simulink model "rocket_multiphase"  (R2024b)
settings: Solver=VariableStepAuto  StartTime=0.0  StopTime=40  RelTol=1e-3
undefined symbols (not defined in the file): K, Kd, Ki, Kp, Tf
libraries: simulink x1, slpidlib x1
settings Model: Creator=fpigh  LastModifiedBy=fpigh

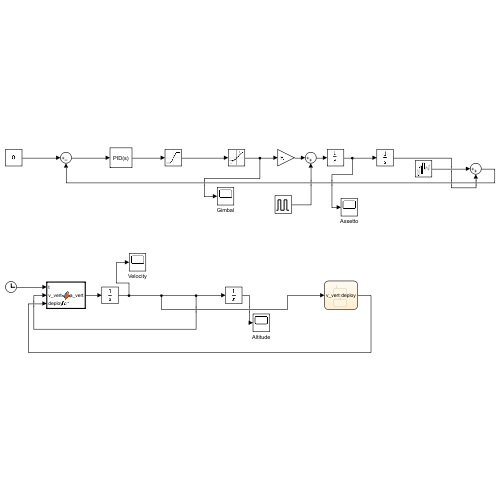
[thumbnail: Simulink's stored preview of the top-level diagram]
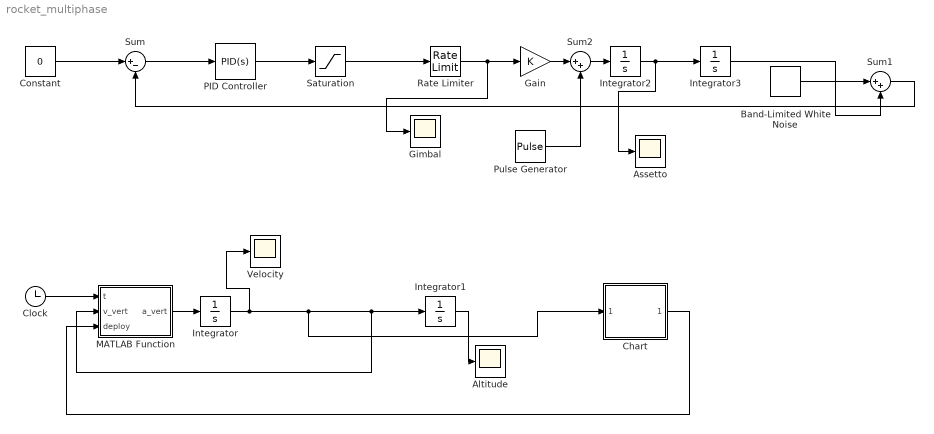
== system rocket_multiphase ==
  Altitude : Scope
  Assetto : Scope
  Band-Limited White Noise : simulink/Sources/Band-Limited White Noise  Cov=1e-9  Ts=0.001  seed=[23341]
  Chart : Stateflow chart  TreatAsAtomicUnit=on
  Clock : Clock
  Constant : Constant  Value=0
  Gain : Gain  Gain=K
  Gimbal : Scope
  Integrator{,1..3} (4 alike) : Integrator
  MATLAB Function : MATLAB Function  TreatAsAtomicUnit=on
  PID Controller : slpidlib/PID Controller  Controller=PID  Form=Parallel  TimeDomain=Continuous-time  UseExternalTs=off  SampleTime=-1  IntegratorMethod=Forward Euler  FilterMethod=Forward Euler  ControllerParametersSource=internal  P=Kp  I=Ki  UseKiTs=off  D=Kd  UseExternalDerivativeSource=off  N=1/Tf  UseFilter=on  TunerSelectOption=Transfer Function Based (PID Tuner App)  InitialConditionSource=internal  InitialConditionForIntegrator=0  InitialConditionForFilter=0  DifferentiatorICPrevScaledInput=0  ExternalReset=none  TrackingMode=off  Kt=1  LimitOutput=off  SatLimitsSource=internal  UpperSaturationLimit=inf  LowerSaturationLimit=-inf  LinearizeAsGain=on  AntiWindupMode=none  Kb=1  LimitIntegrator=off  UpperIntegratorSaturationLimit=inf  LowerIntegratorSaturationLimit=-inf  POutMin=[]  POutMax=[]  IOutMin=[]  IOutMax=[]  DOutMin=[]  DOutMax=[]  NOutMin=[]  NOutMax=[]  SumOutMin=[]  SumOutMax=[]  SaturationOutMin=[]  SaturationOutMax=[]  PParamMin=[]  PParamMax=[]  IParamMin=[]  IParamMax=[]  DParamMin=[]  DParamMax=[]  NParamMin=[]  NParamMax=[]  KbParamMin=[]  KbParamMax=[]  KtParamMin=[]  KtParamMax=[]  KbOutMin=[]  KbOutMax=[]  KtOutMin=[]  KtOutMax=[]  IntegratorOutMin=[]  IntegratorOutMax=[]  FilterOutMin=[]  FilterOutMax=[]  SumI1OutMin=[]  SumI1OutMax=[]  SumI2OutMin=[]  SumI2OutMax=[]  SumI3OutMin=[]  SumI3OutMax=[]  SumI4OutMin=[]  SumI4OutMax=[]  SumDOutMin=[]  SumDOutMax=[]  DifferentiatorOutMin=[]  DifferentiatorOutMax=[]  FilterDiffOutCoefMin=[]  FilterDiffOutCoefMax=[]  ReciprocalOutMin=[]  ReciprocalOutMax=[]  SumDenOutMin=[]  SumDenOutMax=[]  SumNumOutMin=[]  SumNumOutMax=[]  DivideOutMin=[]  DivideOutMax=[]  UdiffTsProdOutMin=[]  UdiffTsProdOutMax=[]  NTsProdOutMin=[]  NTsProdOutMax=[]  UintegralTsProdOutMin=[]  UintegralTsProdOutMax=[]  UngainTsProdOutMin=[]  UngainTsProdOutMax=[]  ClampingZeroOutDataTypeStr=Inherit: Inherit via back propagation  ClampingZeroOutMin=[]  ClampingZeroOutMax=[]  FilterDenConstantOutDataTypeStr=Inherit: Inherit via back propagation  FilterDenConstantOutMin=[]  FilterDenConstantOutMax=[]  PCopyOutDataTypeStr=Inherit: Inherit via back propagation  PCopyOutMin=[]  PCopyOutMax=[]  NCopyOutDataTypeStr=Inherit: Inherit via back propagation  NCopyOutMin=[]  NCopyOutMax=[]  IntegratorContinuousStateAttributes=''  IntegratorStateMustResolveToSignalObject=off  IntegratorRTWStateStorageClass=Auto  FilterContinuousStateAttributes=''  FilterStateMustResolveToSignalObject=off  FilterRTWStateStorageClass=Auto  ParallelPVariant=InternalParameters  IdealPVariant=Disabled  IVariant=InternalParameters  DVariant=InternalParameters  IntegratorVariant=Continuous  SatVariant=Disabled  AWVariant=Passthrough  PCopyVariant=Disabled  TRVariant=Disabled  FdbkBlocksVariant=Forward  IdealPFdbkVariant=Disabled  SatFdbkVariant=Disabled  DerivativeFilterVariant=ContFilter  NVariant=InternalParameters  NCopyVariant=Disabled  FilterICVariant=InternalICsFilter  IntegratorICVariant=InternalICs  ExternalResetVariant=Disabled  TRSumVariant=Passthrough  SumFdbkVariant=Disabled  SumVariant=Sum_PID  TsampFilterVariant=InternalTs  TsampNgainVariant=Passthrough  TsampIntegralVariant=Disabled_SignalSpec  ExternalSaturationOutDataTypeStr=Inherit: Same as second input  DerivativeSourceVariant=ErrorSignal  PreIntVariant=InternalPreInt
  Pulse Generator : DiscretePulseGenerator  PulseType=Time based  Amplitude=5  Period=40  PulseWidth=2  PhaseDelay=3
  Rate Limiter : RateLimiter  RisingSlewLimit=deg2rad(500)  FallingSlewLimit=-deg2rad(500)  SampleTimeMode=inherited
  Saturation : Saturate  UpperLimit=deg2rad(5)  LowerLimit=-deg2rad(5)
  Sum : Sum  Inputs=|+-
  Sum1 : Sum  Inputs=|++
  Sum2 : Sum  Inputs=|++
  Velocity : Scope
  wires:
  Clock/1 -> MATLAB Function/1(t)
  MATLAB Function/1(a_vert) -> Integrator/1
  Integrator/1 -> Velocity/1, Chart/1(v_vert), MATLAB Function/2(v_vert), Integrator1/1
  Integrator1/1 -> Altitude/1
  Chart/1(deploy) -> MATLAB Function/3(deploy)
  Constant/1 -> Sum/1
  Sum/1 -> PID Controller/1
  PID Controller/1 -> Saturation/1
  Saturation/1 -> Rate Limiter/1
  Rate Limiter/1 -> Gimbal/1, Gain/1
  Integrator2/1 -> Assetto/1, Integrator3/1
  Band-Limited White Noise/1 -> Sum1/1
  Integrator3/1 -> Sum1/2
  Sum1/1 -> Sum/2
  Pulse Generator/1 -> Sum2/2
  Gain/1 -> Sum2/1
  Sum2/1 -> Integrator2/1

== stateflow chart rocket_multiphase/Chart ==
  state ASCENT
    entry: deploy = 0;
  state DESCENT
    entry: deploy = 1;
  (default) -> ASCENT
  ASCENT -> DESCENT : [v_vert <= 0]
  data: v_vert input; deploy output

== matlab function rocket_multiphase/MATLAB Function ==
  data: t input; a_vert output; v_vert input; deploy input
function a_vert = fcn(t, v_vert, deploy)
% Dinamica verticale del razzo: restituisce l'accelerazione verticale
% Ingressi:
%   t       = tempo [s]
%   v_vert  = velocità verticale [m/s]
%   deploy  = segnale paracadute (0 = chiuso, 1 = aperto)

%% Parametri (devono combaciare con init_multiphase.m)
m0      = 0.792;    % massa iniziale [kg]
m_dry   = 0.767;    % massa dopo burnout [kg]
t_burn  = 0.99;     % durata spinta [s]
T_avg   = 56;       % spinta media [N]
A_ref   = 22.9e-4;  % area riferimento corpo [m^2]
Cd_asc  = 0.75;     % Cd ascesa
A_para  = pi*(0.70/2)^2;  % area paracadute [m^2]
Cd_para = 0.80;
g       = 9.81;
rho     = 1.225;

%% Spinta e massa (solo durante il burn)
if t < t_burn
    thrust = T_avg;
    mdot   = (m0 - m_dry)/t_burn;
    mass   = m0 - mdot*t;
else
    thrust = 0;
    mass   = m_dry;
end

%% Drag: cambia se il paracadute è aperto
if deploy > 0.5
    drag_area = Cd_para*A_para;   % paracadute aperto
else
    drag_area = Cd_asc*A_ref;     % solo corpo
end
drag = 0.5*rho*v_vert*abs(v_vert)*drag_area;  % si oppone al moto

%% Accelerazione verticale (2a legge di Newton)
a_vert = -g + (thrust - drag)/mass;
